simulink model "Battery_Model_Rint"  (R2025b)
settings: Solver=ode23t  StartTime=0.0  StopTime=1000  MaxStep=0.01  RelTol=1e-4
libraries: fl_lib x6, nesl_utility x6
settings Model: Creator=Ashwin AGGI  LastModifiedBy=psvan

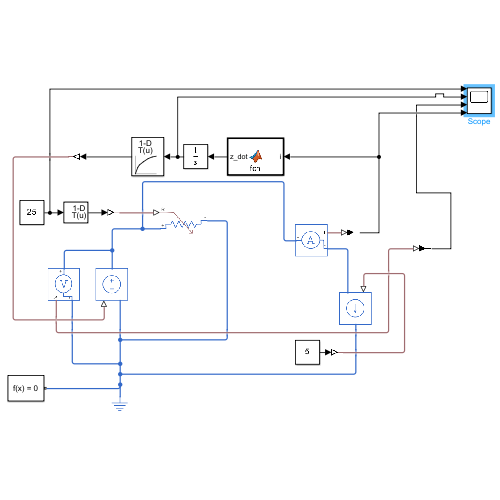
[thumbnail: Simulink's stored preview of the top-level diagram]
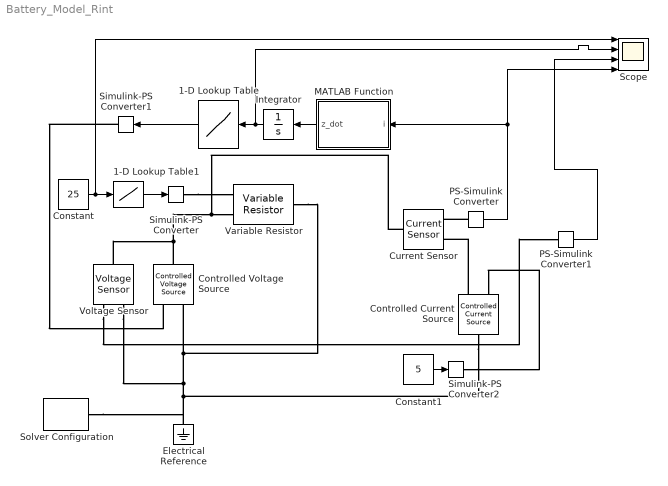
== system Battery_Model_Rint ==
  1-D Lookup Table : Lookup_n-D  NumberOfTableDimensions=1  BreakpointsForDimension1=[0, 0.1, 0.2, 0.4, 0.6, 0.8, 1]  Table=[3.0, 3.4, 3.6, 3.8, 4.0, 4.1, 4.2]  InternalRulePriority=Speed  RndMeth=Simplest
  1-D Lookup Table1 : Lookup_n-D  NumberOfTableDimensions=1  BreakpointsForDimension1=[0,25,40]  Table=[0.019,0.02,0.021]  InternalRulePriority=Speed  RndMeth=Simplest
  Constant : Constant  Value=25
  Constant1 : Constant  Value=5
  Controlled Current Source : fl_lib/Electrical/Electrical Sources/Controlled Current Source
  Controlled Voltage Source : fl_lib/Electrical/Electrical Sources/Controlled Voltage Source
  Current Sensor : fl_lib/Electrical/Electrical Sensors/Current Sensor
  Electrical Reference : fl_lib/Electrical/Electrical Elements/Electrical Reference
  Integrator : Integrator  InitialCondition=0.5
  MATLAB Function : MATLAB Function  TreatAsAtomicUnit=on
  PS-Simulink Converter : nesl_utility/PS-Simulink Converter  PhysicalDomain=network_engine_domain  SubClassName=ps_output  LeftPortType=input  RightPortType=output  PseudoPeriodic=off  Frequencies=[]  VectorFormat=inherit  Unit=inherit  AffineConversion=off
  PS-Simulink Converter1 : nesl_utility/PS-Simulink Converter  PhysicalDomain=network_engine_domain  SubClassName=ps_output  LeftPortType=input  RightPortType=output  PseudoPeriodic=off  Frequencies=[]  VectorFormat=inherit  Unit=inherit  AffineConversion=off
  Scope : Scope  NumInputPorts=4
      settings: SampleTime=1  ActiveDisplayString=3  ActiveDisplayYMinimum=-1.014475754094899  ActiveDisplayYMaximum=6.9191157135233379  YLabel=Terminal Voltage
  Simulink-PS Converter : nesl_utility/Simulink-PS Converter  PhysicalDomain=network_engine_domain  SubClassName=ps_input  LeftPortType=input  RightPortType=output  PseudoPeriodic=off  Frequencies=[]  NoiseDistribution=none  NoiseParameters=[]  Unit=1  AffineConversion=off  FilteringAndDerivatives=provide  SimscapeFilterOrder=1  InputFilterTimeConstant=0.001  UdotUserProvided=0
  Simulink-PS Converter1 : nesl_utility/Simulink-PS Converter  PhysicalDomain=network_engine_domain  SubClassName=ps_input  LeftPortType=input  RightPortType=output  PseudoPeriodic=off  Frequencies=[]  NoiseDistribution=none  NoiseParameters=[]  Unit=1  AffineConversion=off  FilteringAndDerivatives=provide  SimscapeFilterOrder=1  InputFilterTimeConstant=0.001  UdotUserProvided=0
  Simulink-PS Converter2 : nesl_utility/Simulink-PS Converter  PhysicalDomain=network_engine_domain  SubClassName=ps_input  LeftPortType=input  RightPortType=output  PseudoPeriodic=off  Frequencies=[]  NoiseDistribution=none  NoiseParameters=[]  Unit=1  AffineConversion=off  FilteringAndDerivatives=provide  SimscapeFilterOrder=1  InputFilterTimeConstant=0.001  UdotUserProvided=0
  Solver Configuration : nesl_utility/Solver Configuration  PhysicalDomain=network_engine_domain  SubClassName=solver  LeftPortType=input  RightPortType=generic  Tones=[]  Harmonics=[]  SimulateNoise=off  Profile=off  UseLocalSampling=off  EnableSwitchedLinearOptims=on  FrequencyDomain=off  UseCCode=off  RelTol=0.001  AbsTol=0.001  MinStep=1e-09  ToWorkspace=off  RevertToSquareIcSolve=off  NumHomotopyIterations=100  PhasorMode=off  PhasorModeNumHarmonics=1  ConsistencySolver=NEWTON_XTOL_AFTER_FTOL  IndexReductionMethod=DerivativeReplacement  DoDC=off  ResidualTolerance=1e-09  ConsistencyTolSource=GLOBAL  ConsistencyAbsTol=0.001  ConsistencyRelTol=0.001  ConsistencyTolFactor=0.001  UseLocalSolver=off  LocalSolverChoice=NE_BACKWARD_EULER_ADVANCER  ResolveIndetEquations=on  FunctionEvalNumThread=1  LocalSolverSampleTime=0.001  DoFixedCost=off  MaxNonlinIter=3  MaxModeIter=2  ComputeImpulses=off  ImpulseIterations=2  LinearAlgebra=auto  LinearAlgebraNumThread=0  EquationFormulation=NE_TIME_EF  DelaysMemoryBudget=1024  AutomaticFiltering=on  FilteringTimeConstant=0.001  PartitionStorageMethod=AS_NEEDED  PartitionMemoryBudget=1024  PartitionMethod=ROBUST  MultibodyUseLocalSolver=off  MultibodyLocalSolverChoice=ODE1  MultibodyLocalSolverSampleTime=0.001
  Variable Resistor : fl_lib/Electrical/Electrical Elements/Variable Resistor  Rmin=0 Ohm  thermalEnable=false  thermal_mass=1 J/K  i_specify=off  i_priority=None  i=0 A  i_nominal_specify=off  i_nominal_value=1  i_nominal_unit=A  v_specify=off  v_priority=None  v=0 V  v_nominal_specify=off  v_nominal_value=1  v_nominal_unit=V  T_specify=off  T_priority=None  T=300 K  T_nominal_specify=off  T_nominal_value=1  T_nominal_unit=K
  Voltage Sensor : fl_lib/Electrical/Electrical Sensors/Voltage Sensor
  wires:
  MATLAB Function/1(z_dot) -> Integrator/1
  Constant/1 -> Scope/1, 1-D Lookup Table1/1
  1-D Lookup Table1/1 -> Simulink-PS Converter/1
  Integrator/1 -> Scope/2, 1-D Lookup Table/1
  1-D Lookup Table/1 -> Simulink-PS Converter1/1
  PS-Simulink Converter/1 -> Scope/4, MATLAB Function/1(i)
  Constant1/1 -> Simulink-PS Converter2/1
  PS-Simulink Converter1/1 -> Scope/3
  connections:
  Controlled Voltage Source/LConn1 -- Voltage Sensor/LConn1 -- Current Sensor/LConn1 -- Variable Resistor/LConn2
  Variable Resistor/RConn1 -- Controlled Current Source/LConn1 -- Solver Configuration/RConn1 -- Electrical Reference/LConn1 -- Voltage Sensor/RConn2 -- Controlled Voltage Source/RConn2
  Simulink-PS Converter/RConn1 -- Variable Resistor/LConn1
  Simulink-PS Converter1/RConn1 -- Controlled Voltage Source/RConn1
  PS-Simulink Converter/LConn1 -- Current Sensor/RConn1
  Simulink-PS Converter2/RConn1 -- Controlled Current Source/RConn1
  Voltage Sensor/RConn1 -- PS-Simulink Converter1/LConn1
  Controlled Current Source/RConn2 -- Current Sensor/RConn2

== matlab function Battery_Model_Rint/MATLAB Function ==
  data: i input; z_dot output
function z_dot = fcn(i)
% --- Battery Parameters ---
Q = 3600;      % Total capacity in Coulombs (1 Ah)
eta = 0.995;   % Coulombic efficiency

% --- State Equation for SoC ---
z_dot = -(eta * i) / Q;
end
